simulink model "Viz_Logging"  (R2026b)
settings: Solver=VariableStepAuto
undefined symbols (not defined in the file or in its folder): P, shaddad, Ts
settings Model: Creator=aomar  LastModifiedBy=aomar

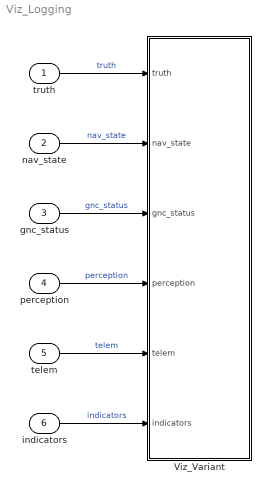
== system Viz_Logging ==
  truth : Inport  OutDataTypeStr=Bus: Bus_TruthState  SampleTime=Ts.base
  nav_state : Inport  Port=2  OutDataTypeStr=Bus: Bus_NavState  SampleTime=Ts.ctrl
  gnc_status : Inport  Port=3  OutDataTypeStr=Bus: Bus_GncStatus  SampleTime=Ts.gnc_status
  perception : Inport  Port=4  OutDataTypeStr=Bus: Bus_Perception  SampleTime=Ts.hk
  telem : Inport  Port=5  OutDataTypeStr=Bus: Bus_FwTelemetry  SampleTime=Ts.ctrl
  indicators : Inport  Port=6  OutDataTypeStr=Bus: Bus_IndicatorOut  SampleTime=Ts.hk
  Viz_Variant : Subsystem  Variant=on
  wires:
  truth/1 -> Viz_Variant/1(truth)  "truth"
  nav_state/1 -> Viz_Variant/2(nav_state)  "nav_state"
  gnc_status/1 -> Viz_Variant/3(gnc_status)  "gnc_status"
  perception/1 -> Viz_Variant/4(perception)  "perception"
  telem/1 -> Viz_Variant/5(telem)  "telem"
  indicators/1 -> Viz_Variant/6(indicators)  "indicators"

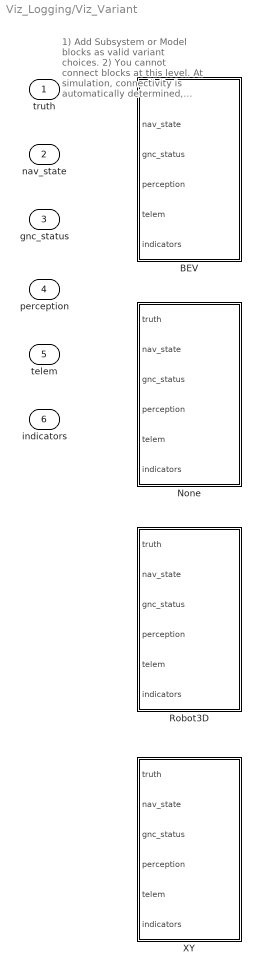
== system Viz_Logging/Viz_Variant ==
  note: 1) Add Subsystem or Model blocks as valid variant choices.
      | 2) You cannot connect blocks at this level. At simulation, connectivity is automatically
      | determined, based on the active variant and port name matching.
  truth : Inport
  nav_state : Inport  Port=2
  gnc_status : Inport  Port=3
  perception : Inport  Port=4
  telem : Inport  Port=5
  indicators : Inport  Port=6
  BEV : Subsystem  Description=VC_VIZ == 1: live bird's-eye view (shaddad.BirdsEyeView, Interpreted execution, 0.1 s).  VariantControl=VC_VIZ == 1
  None : Subsystem  Description=VC_VIZ == 0: no live visualisation.  VariantControl=VC_VIZ == 0
  Robot3D : Subsystem  Description=VC_VIZ == 3: live 3-D view of the robot (shaddad.Robot3DView, Interpreted execution, P.viz.Ts3d): body, moving tracks, implement, follow camera, HUD, Stop button.  VariantControl=VC_VIZ == 3
  XY : Subsystem  Description=VC_VIZ == 2: XY Graph of the truth and NavState positions (0.1 s).  VariantControl=VC_VIZ == 2

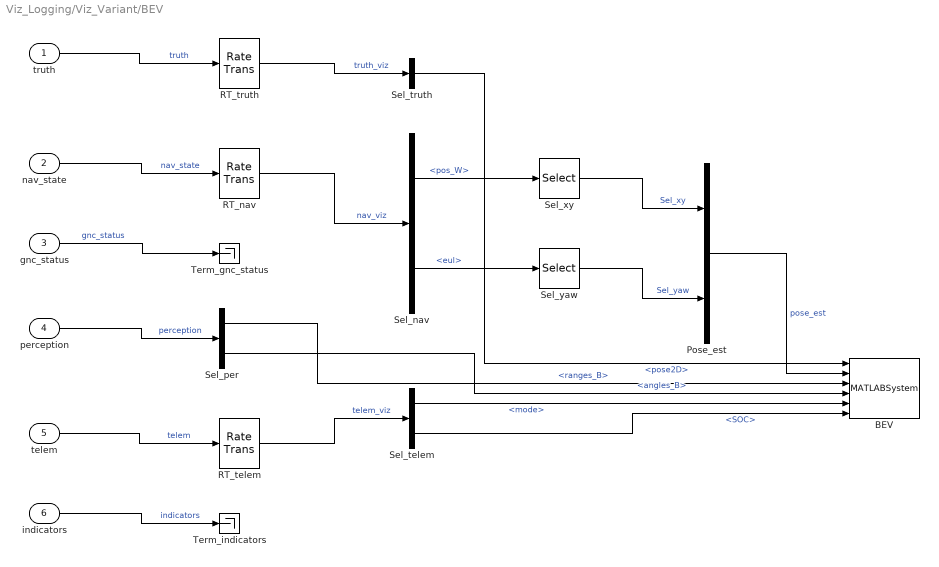
== system Viz_Logging/Viz_Variant/BEV ==
  truth : Inport  OutDataTypeStr=Bus: Bus_TruthState
  nav_state : Inport  Port=2  OutDataTypeStr=Bus: Bus_NavState
  gnc_status : Inport  Port=3  OutDataTypeStr=Bus: Bus_GncStatus
  perception : Inport  Port=4  OutDataTypeStr=Bus: Bus_Perception
  telem : Inport  Port=5  OutDataTypeStr=Bus: Bus_FwTelemetry
  indicators : Inport  Port=6  OutDataTypeStr=Bus: Bus_IndicatorOut
  BEV : MATLABSystem  System=shaddad.BirdsEyeView  MapImage=P.world.occ.grid  MapResolution=P.world.occ.res  MapOrigin=P.world.occ.origin  Footprint=P.viz.footprint  TrailLength=P.viz.trail_len  ScanDecim=P.viz.scan_decim  SampleTime=P.viz.Ts  PathXY=shaddad.BirdsEyeView.planPath(P.gnc.mission)  Visible=true
      mask Type: shaddad.BirdsEyeView
  Pose_est : Concatenate
  RT_nav : RateTransition  InitialCondition=P.ic.Bus_NavState  OutPortSampleTime=P.viz.Ts
  RT_telem : RateTransition  InitialCondition=P.ic.Bus_FwTelemetry  OutPortSampleTime=P.viz.Ts
  RT_truth : RateTransition  InitialCondition=P.ic.Bus_TruthState  OutPortSampleTime=P.viz.Ts
  Sel_nav : BusSelector  OutputSignals=pos_W,eul
  Sel_per : BusSelector  OutputSignals=ranges_B,angles_B
  Sel_telem : BusSelector  OutputSignals=mode,SOC
  Sel_truth : BusSelector  OutputSignals=pose2D
  Sel_xy : Selector  InputPortWidth=3  IndexOptions=Index vector (dialog)  Indices=[1 2]  OutputSizes=1
  Sel_yaw : Selector  InputPortWidth=3  IndexOptions=Index vector (dialog)  Indices=1  OutputSizes=1
  Term_gnc_status : Terminator
  Term_indicators : Terminator
  wires:
  truth/1 -> RT_truth/1  "truth"
  nav_state/1 -> RT_nav/1  "nav_state"
  gnc_status/1 -> Term_gnc_status/1  "gnc_status"
  perception/1 -> Sel_per/1  "perception"
  telem/1 -> RT_telem/1  "telem"
  indicators/1 -> Term_indicators/1  "indicators"
  Sel_per/1 -> BEV/3  "<ranges_B>"
  Sel_per/2 -> BEV/4  "<angles_B>"
  RT_truth/1 -> Sel_truth/1  "truth_viz"
  RT_nav/1 -> Sel_nav/1  "nav_viz"
  RT_telem/1 -> Sel_telem/1  "telem_viz"
  Sel_truth/1 -> BEV/1  "<pose2D>"
  Sel_nav/1 -> Sel_xy/1  "<pos_W>"
  Sel_nav/2 -> Sel_yaw/1  "<eul>"
  Sel_telem/1 -> BEV/5  "<mode>"
  Sel_telem/2 -> BEV/6  "<SOC>"
  Sel_xy/1 -> Pose_est/1  "Sel_xy"
  Sel_yaw/1 -> Pose_est/2  "Sel_yaw"
  Pose_est/1 -> BEV/2  "pose_est"

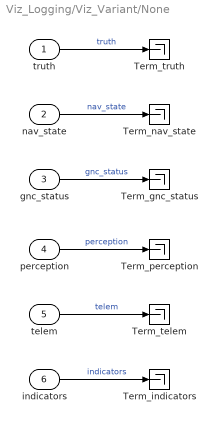
== system Viz_Logging/Viz_Variant/None ==
  truth : Inport  OutDataTypeStr=Bus: Bus_TruthState
  nav_state : Inport  Port=2  OutDataTypeStr=Bus: Bus_NavState
  gnc_status : Inport  Port=3  OutDataTypeStr=Bus: Bus_GncStatus
  perception : Inport  Port=4  OutDataTypeStr=Bus: Bus_Perception
  telem : Inport  Port=5  OutDataTypeStr=Bus: Bus_FwTelemetry
  indicators : Inport  Port=6  OutDataTypeStr=Bus: Bus_IndicatorOut
  Term_gnc_status : Terminator
  Term_indicators : Terminator
  Term_nav_state : Terminator
  Term_perception : Terminator
  Term_telem : Terminator
  Term_truth : Terminator
  wires:
  truth/1 -> Term_truth/1  "truth"
  nav_state/1 -> Term_nav_state/1  "nav_state"
  gnc_status/1 -> Term_gnc_status/1  "gnc_status"
  perception/1 -> Term_perception/1  "perception"
  telem/1 -> Term_telem/1  "telem"
  indicators/1 -> Term_indicators/1  "indicators"

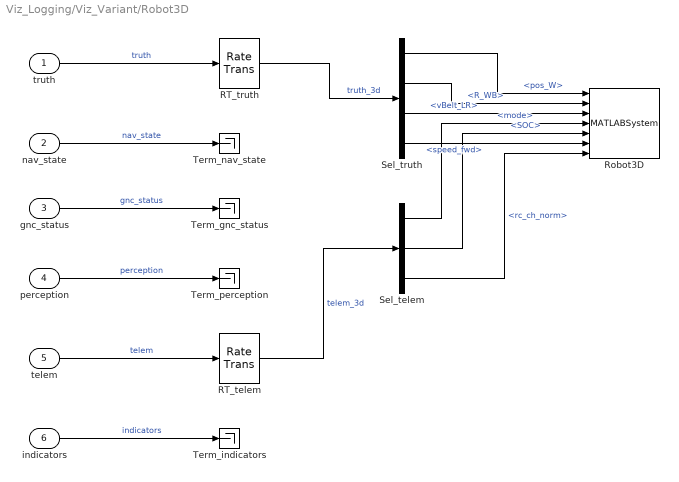
== system Viz_Logging/Viz_Variant/Robot3D ==
  truth : Inport  OutDataTypeStr=Bus: Bus_TruthState
  nav_state : Inport  Port=2  OutDataTypeStr=Bus: Bus_NavState
  gnc_status : Inport  Port=3  OutDataTypeStr=Bus: Bus_GncStatus
  perception : Inport  Port=4  OutDataTypeStr=Bus: Bus_Perception
  telem : Inport  Port=5  OutDataTypeStr=Bus: Bus_FwTelemetry
  indicators : Inport  Port=6  OutDataTypeStr=Bus: Bus_IndicatorOut
  RT_telem : RateTransition  InitialCondition=P.ic.Bus_FwTelemetry  OutPortSampleTime=P.viz.Ts3d
  RT_truth : RateTransition  InitialCondition=P.ic.Bus_TruthState  OutPortSampleTime=P.viz.Ts3d
  Robot3D : MATLABSystem  System=shaddad.Robot3DView  Implement=VC_IMPL  SampleTime=P.viz.Ts3d  Camera=P.viz.camera  ModelName=Shaddad_System  Obstacles=[ 0, 0, 0 ]  Visible=true
      mask Type: shaddad.Robot3DView
  Sel_telem : BusSelector  OutputSignals=mode,SOC,rc_ch_norm
  Sel_truth : BusSelector  OutputSignals=pos_W,R_WB,vBelt_LR,speed_fwd
  Term_gnc_status : Terminator
  Term_indicators : Terminator
  Term_nav_state : Terminator
  Term_perception : Terminator
  wires:
  truth/1 -> RT_truth/1  "truth"
  nav_state/1 -> Term_nav_state/1  "nav_state"
  gnc_status/1 -> Term_gnc_status/1  "gnc_status"
  perception/1 -> Term_perception/1  "perception"
  telem/1 -> RT_telem/1  "telem"
  indicators/1 -> Term_indicators/1  "indicators"
  RT_truth/1 -> Sel_truth/1  "truth_3d"
  RT_telem/1 -> Sel_telem/1  "telem_3d"
  Sel_truth/1 -> Robot3D/1  "<pos_W>"
  Sel_truth/2 -> Robot3D/2  "<R_WB>"
  Sel_truth/3 -> Robot3D/3  "<vBelt_LR>"
  Sel_truth/4 -> Robot3D/6  "<speed_fwd>"
  Sel_telem/1 -> Robot3D/4  "<mode>"
  Sel_telem/2 -> Robot3D/5  "<SOC>"
  Sel_telem/3 -> Robot3D/7  "<rc_ch_norm>"

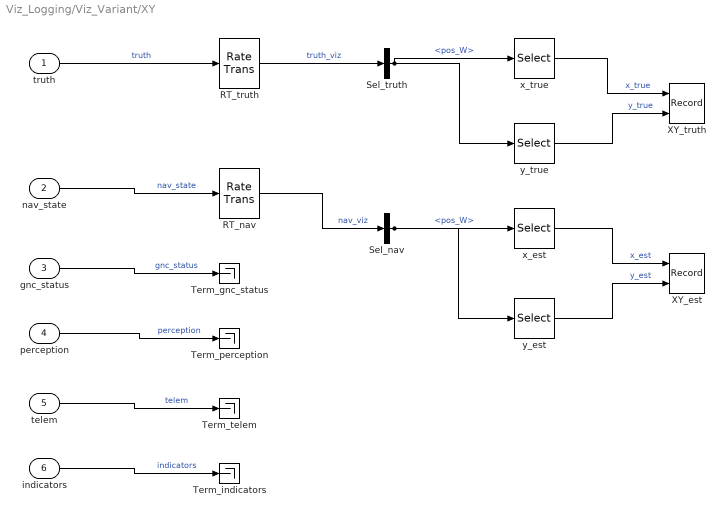
== system Viz_Logging/Viz_Variant/XY ==
  truth : Inport  OutDataTypeStr=Bus: Bus_TruthState
  nav_state : Inport  Port=2  OutDataTypeStr=Bus: Bus_NavState
  gnc_status : Inport  Port=3  OutDataTypeStr=Bus: Bus_GncStatus
  perception : Inport  Port=4  OutDataTypeStr=Bus: Bus_Perception
  telem : Inport  Port=5  OutDataTypeStr=Bus: Bus_FwTelemetry
  indicators : Inport  Port=6  OutDataTypeStr=Bus: Bus_IndicatorOut
  RT_nav : RateTransition  InitialCondition=P.ic.Bus_NavState  OutPortSampleTime=P.viz.Ts
  RT_truth : RateTransition  InitialCondition=P.ic.Bus_TruthState  OutPortSampleTime=P.viz.Ts
  Sel_nav : BusSelector  OutputSignals=pos_W
  Sel_truth : BusSelector  OutputSignals=pos_W
  Term_gnc_status : Terminator
  Term_indicators : Terminator
  Term_perception : Terminator
  Term_telem : Terminator
  XY_est : Record  NumPorts=2.0  FileSettingsInternal="{\"entries\":[{\"content\":{\"excelSettings\":{\"content\":{},\"type\":\"Streamout.ExcelSettings\"},\"parquetSettings\":{\"content\":{},\"type\":\"Streamout.ParquetSettings\"}},\"type\":\"Streamout.FileSettingStorage\",\"uuid\":\"\"}],\"packageUris\":[\"http:\\/\\/schema.mathworks.com\\/mf0\\/streamout_blocks\\/R2020a\"],\"version\":\"1.0\"}"  FrameSettings=[0, 0]  Layout=[1 1]  SignalsInternal="{\"entries\":[{\"content\":{\"signals\":[{\"content\":{\"blockPath\":[],\"dimensions\":[1],\"domain\":\"\",\"lineColor\":\"#a2142f\",\"plots\":[ 1 ],\"port\":1,\"signalID\":1,\"signalName\":\"XY Graph:1\"},\"type\":\"RecordBlkView.Signal\",\"uuid\":\"\"},{\"content\":{\"blockPath\":[],\"dimensions\":[1],\"domain\":\"\",\"lineColor\":\"#139fff\",\"plots\":[ 1 ],\"port\":2,\"signalID\":2,\"signalName\":\"XY Graph:2\"},\"type\":\"RecordBlkView.Signal\",\"uuid\":\"\"}]},\"type\":\"RecordBlkView.InputSignals\",\"uuid\":\"\"}],\"packageUris\":[\"http:\\/\\/schema.mathworks.com\\/mf0\\/streamout_blocks\\/R2020a\"],\"version\":\"1.0\"}"  VisualizationBindings="{\"xyplotplugin\":{\"info\":[{\"series\":[{\"bindingParametersList\":[{\"parameter\":\"X-Axis\",\"signalID\":1,\"signalName\":\"XY Graph:1\"},{\"parameter\":\"Y-Axis\",\"signalID\":2,\"signalName\":\"XY Graph:2\"}],\"seriesID\":0}],\"subplotID\":1}]}}"  CompatibilityTag=XY
  XY_truth : Record  NumPorts=2.0  FileSettingsInternal="{\"entries\":[{\"content\":{\"excelSettings\":{\"content\":{},\"type\":\"Streamout.ExcelSettings\"},\"parquetSettings\":{\"content\":{},\"type\":\"Streamout.ParquetSettings\"}},\"type\":\"Streamout.FileSettingStorage\",\"uuid\":\"\"}],\"packageUris\":[\"http:\\/\\/schema.mathworks.com\\/mf0\\/streamout_blocks\\/R2020a\"],\"version\":\"1.0\"}"  FrameSettings=[0, 0]  Layout=[1 1]  SignalsInternal="{\"entries\":[{\"content\":{\"signals\":[{\"content\":{\"blockPath\":[],\"dimensions\":[1],\"domain\":\"\",\"lineColor\":\"#a2142f\",\"plots\":[ 1 ],\"port\":1,\"signalID\":1,\"signalName\":\"XY Graph:1\"},\"type\":\"RecordBlkView.Signal\",\"uuid\":\"\"},{\"content\":{\"blockPath\":[],\"dimensions\":[1],\"domain\":\"\",\"lineColor\":\"#139fff\",\"plots\":[ 1 ],\"port\":2,\"signalID\":2,\"signalName\":\"XY Graph:2\"},\"type\":\"RecordBlkView.Signal\",\"uuid\":\"\"}]},\"type\":\"RecordBlkView.InputSignals\",\"uuid\":\"\"}],\"packageUris\":[\"http:\\/\\/schema.mathworks.com\\/mf0\\/streamout_blocks\\/R2020a\"],\"version\":\"1.0\"}"  VisualizationBindings="{\"xyplotplugin\":{\"info\":[{\"series\":[{\"bindingParametersList\":[{\"parameter\":\"X-Axis\",\"signalID\":1,\"signalName\":\"XY Graph:1\"},{\"parameter\":\"Y-Axis\",\"signalID\":2,\"signalName\":\"XY Graph:2\"}],\"seriesID\":0}],\"subplotID\":1}]}}"  CompatibilityTag=XY
  x_est : Selector  InputPortWidth=3  IndexOptions=Index vector (dialog)  Indices=1  OutputSizes=1
  x_true : Selector  InputPortWidth=3  IndexOptions=Index vector (dialog)  Indices=1  OutputSizes=1
  y_est : Selector  InputPortWidth=3  IndexOptions=Index vector (dialog)  Indices=2  OutputSizes=1
  y_true : Selector  InputPortWidth=3  IndexOptions=Index vector (dialog)  Indices=2  OutputSizes=1
  wires:
  truth/1 -> RT_truth/1  "truth"
  nav_state/1 -> RT_nav/1  "nav_state"
  gnc_status/1 -> Term_gnc_status/1  "gnc_status"
  perception/1 -> Term_perception/1  "perception"
  telem/1 -> Term_telem/1  "telem"
  indicators/1 -> Term_indicators/1  "indicators"
  RT_truth/1 -> Sel_truth/1  "truth_viz"
  RT_nav/1 -> Sel_nav/1  "nav_viz"
  Sel_truth/1 -> y_true/1, x_true/1  "<pos_W>"
  Sel_nav/1 -> y_est/1, x_est/1  "<pos_W>"
  x_true/1 -> XY_truth/1  "x_true"
  y_true/1 -> XY_truth/2  "y_true"
  x_est/1 -> XY_est/1  "x_est"
  y_est/1 -> XY_est/2  "y_est"
